simulink model "powertrain_model"  (R2025a)
settings: Solver=ode23tb  StartTime=0.0  StopTime=simlength  FixedStep=tc  MaxStep=tc
values from neighbouring files (symbols this model uses):
  angle_error = angle_error_deg/180*pi    (= 0)    [init_model.m]
  CTRPIFF_CLIP_RELEASE = 0.001    [init_model.m]
  dead_time = dead_time_INV    (= 4.2e-07)    [init_model.m]
  dead_time_INV = 0.42e-6    (= 4.2e-07)    [init_model.m]
  DThs_init = 0    [init_model.m]
  emf_fb_p = 0.2    [init_model.m]
  emf_fb_p_ccaller_1 = emf_fb_p    (= 0.2)    [init_model.m]
  emf_fb_p_ccaller_2 = emf_fb_p    (= 0.2)    [init_model.m]
  emf_p = emf_fb_p*4/10    (= 0.08)    [init_model.m]
  emf_p_ccaller_1 = emf_fb_p_ccaller_1*4/10    (= 0.08)    [init_model.m]
  emf_p_ccaller_2 = emf_fb_p_ccaller_2*4/10    (= 0.08)    [init_model.m]
  fPWM_INV = 25e3    (= 25000)    [init_model.m]
  g0_reference_flt = fcut_reference_flt * ts_inv * 2*pi    (= 0.00100530964915)    [init_model.m]
  g1_reference_flt = 1 - g0_reference_flt    (= 0.998994690351)    [init_model.m]
  id_ref_if_pu = iload_rms_ref*sqrt(2)/ibez    [init_model.m]
  kalman_omega = kw    [init_model.m]
  kalman_theta = kg    [init_model.m]
  kg = K(1)    [init_model.m]
  ki_id = 2    [analysis_cc.m]    (also in init_model.m = 9)
  ki_iq = 9    [init_model.m]
  ki_w = 1    [init_model.m]
  kp_id = 0.15    [analysis_cc.m]    (also in init_model.m = 0.25)
  kp_iq = 0.2    [init_model.m]
  kp_w = 1    [init_model.m]
  kw = K(2)    [init_model.m]
  luenberger_l1 = Klo(1)    [init_model.m]
  luenberger_l2 = Klo(2)    [init_model.m]
  luenberger_l3 = Klo(3)    [init_model.m]
  motorc_m_scale = 2/3*Vdc_bez/ubez    [init_model.m]
  number_of_cells = 100    [init_model.m]
  omega_flt_fcut = 10    [init_model.m]
  omega_flt_g0 = omega_flt_fcut * ts_inv * 2*pi    (= 0.00251327412287)    [init_model.m]
  omega_flt_g1 = 1 - omega_flt_g0    (= 0.997486725877)    [init_model.m]
  omega_ref_if_pu = 1200*2*pi/omega_bez    [init_model.m]
  phase_compensation_omega = 0    [init_model.m]
  pwm_out_lim = 1    [init_model.m]
  Q = 10    [init_model.m]
  q1Kalman = ts_inv^2    (= 1.6e-09)    [init_model.m]
  q2Kalman = ts_inv^1    (= 4e-05)    [init_model.m]
  q3Kalman = 0    [init_model.m]
  rKalman = 1    [init_model.m]
  Tambient = 1    [init_model.m]
  tc = ts_inv/200    (= 2e-07)    [init_model.m]
  time_init = 0.025    [init_model.m]
  torque_ref = 64/ibez*torque_mode    [init_model.m]
  ts_inv = 1/fPWM_INV    (= 4e-05)    [init_model.m]
  tsample = ts_inv    (= 4e-05)    [init_model.m]
  u_flt_g0 = u_flt_fcut * ts_inv * 2*pi    (= 0.904778684234)    [init_model.m]
  u_flt_g1 = 1 - u_flt_g0    (= 0.0952213157661)    [init_model.m]
  Vdc_bez = 400    [init_model.m]
undefined symbols (not defined in the file or in its folder): b, ibez, Jm, Jm_norm, Ld_norm, Lq_norm, Ls_norm, magnitude, omega_bez, psi_bez, psi_m, psi_m_norm, R_RLload, Rload_eq, Rs_norm, tau_bez, weigth
libraries: fl_lib x100, nesl_utility x84, ee_lib x11, cstblocks x4, lithium_ion_cell_lib x1, simulink x1, pmsm_uvw_with_harmonics_lib x1, pmsm_spatial_harmonics_uvw_lib x1, flexshaft_lib x1
(part 5 of 6)

== system powertrain_model/battery_system/battery_system/LithiumIonBattery/lithium ion cell analytical ocv/white_noise ==
  in : Inport
  Band-Limited White Noise : simulink/Sources/Band-Limited White Noise  Commented=on  Cov=tsample  Ts=tsample  seed=[23341]
  Sum2 : Sum  Inputs=|++
  out : Outport
  wires:
  Band-Limited White Noise/1 -> Sum2/2
  Sum2/1 -> out/1
  in/1 -> Sum2/1

== system powertrain_model/driver control/current_ctrl/vector_current_ctrl/dq_vector_pi/bounder1 ==
  md : Inport
  m_1 : Inport  Port=2
  m : Inport  Port=3
  Constant : Constant
  Constant1 : Constant  Value=0
  Divide : Product
  Switch : Switch  Threshold=pwm_out_lim  SaturateOnIntegerOverflow=off  InputSameDT=off
  Switch1 : Switch  Threshold=pwm_out_lim  SaturateOnIntegerOverflow=off  InputSameDT=off
  md_sat : Outport  VectorParamsAs1DForOutWhenUnconnected=off
  clip : Outport  Port=2  VectorParamsAs1DForOutWhenUnconnected=off
  wires:
  md/1 -> Switch1/3, Divide/2
  m_1/1 -> Divide/1
  Divide/1 -> Switch1/1
  Switch1/1 -> md_sat/1
  Switch/1 -> clip/1
  m/1 -> Switch/2, Switch1/2
  Constant/1 -> Switch/1
  Constant1/1 -> Switch/3

== system powertrain_model/driver control/current_ctrl/vector_current_ctrl/dq_vector_pi/bounder2 ==
  m : Inport
  m_1 : Inport  Port=2
  mq : Inport  Port=3
  Constant : Constant
  Constant1 : Constant  Value=0
  Divide : Product
  Switch : Switch  Threshold=pwm_out_lim  SaturateOnIntegerOverflow=off  InputSameDT=off
  Switch1 : Switch  Threshold=pwm_out_lim  SaturateOnIntegerOverflow=off  InputSameDT=off
  mq_sat : Outport  VectorParamsAs1DForOutWhenUnconnected=off
  clip : Outport  Port=2  VectorParamsAs1DForOutWhenUnconnected=off
  wires:
  Constant1/1 -> Switch/3
  Constant/1 -> Switch/1
  m/1 -> Switch1/2, Switch/2
  Switch/1 -> clip/1
  Switch1/1 -> mq_sat/1
  Divide/1 -> Switch1/1
  m_1/1 -> Divide/1
  mq/1 -> Divide/2, Switch1/3

== system powertrain_model/driver control/current_ctrl/vector_current_ctrl/dq_vector_pi/pi_d ==
  id_tilde : Inport
  clip : Inport  Port=2
  1/Ti : Gain  Gain=kp_id  SaturateOnIntegerOverflow=on  OutDataTypeStr=Inherit: Same as input  ParamDataTypeStr=Inherit: Same as input
  Constant : Constant  Value=0
  Constant1 : Constant  Value=Ls_norm
  Product : Product  Inputs=3
  Sum2 : Sum  Inputs=+-  SaturateOnIntegerOverflow=on
  Sum4 : Sum  SaturateOnIntegerOverflow=on
  Sum5 : Sum  Inputs=+++  SaturateOnIntegerOverflow=on
  Switch1 : Switch  Threshold=0.5  SaturateOnIntegerOverflow=off  InputSameDT=off
  Switch2 : Switch  Threshold=0.5  SaturateOnIntegerOverflow=off  InputSameDT=off
  Unit Delay1 : UnitDelay  SampleTime=ts_inv  HasFrameUpgradeWarning=on
  Unit Delay2 : UnitDelay  SampleTime=ts_inv  HasFrameUpgradeWarning=on
  kp1 : Gain  Gain=CTRPIFF_CLIP_RELEASE*ts_inv  SaturateOnIntegerOverflow=on  OutDataTypeStr=Inherit: Same as input  ParamDataTypeStr=Inherit: Same as input
  kp2 : Gain  Gain=ki_id*ts_inv  SaturateOnIntegerOverflow=on  OutDataTypeStr=Inherit: Same as input  ParamDataTypeStr=Inherit: Same as input
  kp3 : Gain  Gain=0  SaturateOnIntegerOverflow=on  OutDataTypeStr=Inherit: Same as input  ParamDataTypeStr=Inherit: Same as input
  ud_out : Outport  VectorParamsAs1DForOutWhenUnconnected=off
  wires:
  id_tilde/1 -> kp2/1, 1/Ti/1
  Switch1/1 -> Unit Delay2/1
  Sum4/1 -> Sum5/2, Switch1/3
  kp1/1 -> Sum2/2
  Sum2/1 -> Switch1/1
  Unit Delay2/1 -> Sum4/2, kp1/1, Sum2/1
  1/Ti/1 -> Sum5/1
  Switch2/1 -> Sum4/1
  kp2/1 -> Switch2/3
  clip/1 -> Unit Delay1/1
  [clip] -> Switch2/2
  [clip] -> Switch1/2
  Constant/1 -> Switch2/1
  Unit Delay1/1 -> [clip]
  Sum5/1 -> ud_out/1
  [iq_inverter_pu] -> Product/2
  [omega_pu_hat_flt] -> Product/1
  kp3/1 -> Sum5/3
  Constant1/1 -> Product/3
  Product/1 -> kp3/1

== system powertrain_model/driver control/current_ctrl/vector_current_ctrl/dq_vector_pi/pi_q ==
  iq_tilde : Inport
  clip : Inport  Port=2
  1/Ti : Gain  Gain=kp_iq  SaturateOnIntegerOverflow=on  OutDataTypeStr=Inherit: Same as input  ParamDataTypeStr=Inherit: Same as input
  Constant : Constant  Value=0
  Constant1 : Constant  Value=Ls_norm
  Product : Product  Inputs=3
  Sum2 : Sum  Inputs=+-  SaturateOnIntegerOverflow=on
  Sum4 : Sum  SaturateOnIntegerOverflow=on
  Sum5 : Sum  Inputs=+++  SaturateOnIntegerOverflow=on
  Switch1 : Switch  Threshold=0.5  SaturateOnIntegerOverflow=off  InputSameDT=off
  Switch2 : Switch  Threshold=0.5  SaturateOnIntegerOverflow=off  InputSameDT=off
  Unit Delay1 : UnitDelay  SampleTime=ts_inv  HasFrameUpgradeWarning=on
  Unit Delay2 : UnitDelay  SampleTime=ts_inv  HasFrameUpgradeWarning=on
  kp1 : Gain  Gain=CTRPIFF_CLIP_RELEASE*ts_inv  SaturateOnIntegerOverflow=on  OutDataTypeStr=Inherit: Same as input  ParamDataTypeStr=Inherit: Same as input
  kp2 : Gain  Gain=ki_iq*ts_inv  SaturateOnIntegerOverflow=on  OutDataTypeStr=Inherit: Same as input  ParamDataTypeStr=Inherit: Same as input
  kp3 : Gain  Gain=0  SaturateOnIntegerOverflow=on  OutDataTypeStr=Inherit: Same as input  ParamDataTypeStr=Inherit: Same as input
  Vqs_out : Outport  VectorParamsAs1DForOutWhenUnconnected=off
  wires:
  Constant/1 -> Switch2/1
  [clip] -> Switch1/2
  [clip] -> Switch2/2
  clip/1 -> Unit Delay1/1
  kp2/1 -> Switch2/3
  Switch2/1 -> Sum4/1
  1/Ti/1 -> Sum5/1
  Unit Delay2/1 -> Sum2/1, kp1/1, Sum4/2
  Sum2/1 -> Switch1/1
  kp1/1 -> Sum2/2
  Sum4/1 -> Sum5/2, Switch1/3
  Switch1/1 -> Unit Delay2/1
  iq_tilde/1 -> 1/Ti/1, kp2/1
  Unit Delay1/1 -> [clip]
  Sum5/1 -> Vqs_out/1
  [omega_pu_hat_flt] -> Product/1
  [id_inverter_pu] -> Product/2
  Constant1/1 -> Product/3
  Product/1 -> kp3/1
  kp3/1 -> Sum5/3

== system powertrain_model/driver control/current_ctrl/vector_current_ctrl/dq_vector_pi/switch ==
  clip 1 : Inport
  clip 2 : Inport  Port=2
  Constant4 : Constant
  Constant5 : Constant  Value=0
  Sum1 : Sum  SaturateOnIntegerOverflow=on
  Switch : Switch  Threshold=0.5  SaturateOnIntegerOverflow=off  InputSameDT=off
  clip : Outport  VectorParamsAs1DForOutWhenUnconnected=off
  wires:
  Constant5/1 -> Switch/3
  Switch/1 -> clip/1
  Constant4/1 -> Switch/1
  Sum1/1 -> Switch/2
  clip 1/1 -> Sum1/1
  clip 2/1 -> Sum1/2

== system powertrain_model/driver control/current_ctrl/vector_current_ctrl/dq_vector_pi/vector lenght ==
  md : Inport
  mq : Inport  Port=2
  Math Function : Math  Operator=magnitude^2  SignedPower=on
  Math Function1 : Math  Operator=magnitude^2  SignedPower=on
  Math Function2 : Math  Operator=reciprocal  SignedPower=on
  Sqrt : Sqrt
  Sum5 : Sum  SaturateOnIntegerOverflow=on
  m_1 : Outport  VectorParamsAs1DForOutWhenUnconnected=off
  m : Outport  Port=2  VectorParamsAs1DForOutWhenUnconnected=off
  wires:
  Sqrt/1 -> m/1, Math Function2/1
  mq/1 -> Math Function1/1
  Math Function1/1 -> Sum5/2
  Math Function/1 -> Sum5/1
  Sum5/1 -> Sqrt/1
  Math Function2/1 -> m_1/1
  md/1 -> Math Function/1

== system powertrain_model/driver control/current_ctrl/vector_current_ctrl/dq_vector_pi_ccaller/Reset Trigger ==
  Step : Step  Time=time_init  Before=1  After=0  SampleTime=0
  Out1 : Outport
  wires:
  Step/1 -> Out1/1  "Reset"

== system powertrain_model/inverter/MOS based inverter/inverter/inverter_mosfet_leg_thermal/mosfet_3 ==
  Diode : fl_lib/Electrical/Electrical Elements/Diode  Vf=Vgamma V  Ron=Ron Ohm  Goff=1e-8 1/Ohm  i_specify=off  i_priority=None  i=0 A  i_nominal_specify=off  i_nominal_value=1  i_nominal_unit=A  v_specify=off  v_priority=None  v=0 V  v_nominal_specify=off  v_nominal_value=1  v_nominal_unit=V
  Switch : fl_lib/Electrical/Electrical Elements/Switch  R_closed=Ron Ohm  G_open=1e-8 1/Ohm  Threshold=7.5  i_specify=off  i_priority=None  i=0 A  i_nominal_specify=off  i_nominal_value=1  i_nominal_unit=A  v_specify=off  v_priority=None  v=0 V  v_nominal_specify=off  v_nominal_value=1  v_nominal_unit=V
  G : PMIOPort  Side=Left
  C : PMIOPort  Port=2  Side=Left
  E : PMIOPort  Port=3  Side=Right
  connections:
  Diode/LConn1 -- E/RConn1 -- Switch/LConn1
  Switch/RConn1 -- G/RConn1
  Diode/RConn1 -- C/RConn1 -- Switch/RConn2

== system powertrain_model/inverter/MOS based inverter/inverter/inverter_mosfet_leg_thermal/mosfet_4 ==
  Diode : fl_lib/Electrical/Electrical Elements/Diode  Vf=Vgamma V  Ron=Ron Ohm  Goff=1e-8 1/Ohm  i_specify=off  i_priority=None  i=0 A  i_nominal_specify=off  i_nominal_value=1  i_nominal_unit=A  v_specify=off  v_priority=None  v=0 V  v_nominal_specify=off  v_nominal_value=1  v_nominal_unit=V
  Switch : fl_lib/Electrical/Electrical Elements/Switch  R_closed=Ron Ohm  G_open=1e-8 1/Ohm  Threshold=7.5  i_specify=off  i_priority=None  i=0 A  i_nominal_specify=off  i_nominal_value=1  i_nominal_unit=A  v_specify=off  v_priority=None  v=0 V  v_nominal_specify=off  v_nominal_value=1  v_nominal_unit=V
  G : PMIOPort  Side=Left
  C : PMIOPort  Port=2  Side=Left
  E : PMIOPort  Port=3  Side=Right
  connections:
  Switch/RConn2 -- C/RConn1 -- Diode/RConn1
  Switch/RConn1 -- G/RConn1
  Switch/LConn1 -- E/RConn1 -- Diode/LConn1

== system powertrain_model/inverter/MOS based inverter/inverter/inverter_mosfet_leg_thermal/mosfet_5 ==
  Diode : fl_lib/Electrical/Electrical Elements/Diode  Vf=Vgamma V  Ron=Ron Ohm  Goff=1e-8 1/Ohm  i_specify=off  i_priority=None  i=0 A  i_nominal_specify=off  i_nominal_value=1  i_nominal_unit=A  v_specify=off  v_priority=None  v=0 V  v_nominal_specify=off  v_nominal_value=1  v_nominal_unit=V
  Switch : fl_lib/Electrical/Electrical Elements/Switch  R_closed=Ron Ohm  G_open=1e-8 1/Ohm  Threshold=7.5  i_specify=off  i_priority=None  i=0 A  i_nominal_specify=off  i_nominal_value=1  i_nominal_unit=A  v_specify=off  v_priority=None  v=0 V  v_nominal_specify=off  v_nominal_value=1  v_nominal_unit=V
  G : PMIOPort  Side=Left
  C : PMIOPort  Port=2  Side=Left
  E : PMIOPort  Port=3  Side=Right
  connections:
  Diode/LConn1 -- E/RConn1 -- Switch/LConn1
  Switch/RConn1 -- G/RConn1
  Diode/RConn1 -- C/RConn1 -- Switch/RConn2

== system powertrain_model/inverter/MOS based inverter/inverter/inverter_mosfet_leg_thermal/mosfet_6 ==
  Diode : fl_lib/Electrical/Electrical Elements/Diode  Vf=Vgamma V  Ron=Ron Ohm  Goff=1e-8 1/Ohm  i_specify=off  i_priority=None  i=0 A  i_nominal_specify=off  i_nominal_value=1  i_nominal_unit=A  v_specify=off  v_priority=None  v=0 V  v_nominal_specify=off  v_nominal_value=1  v_nominal_unit=V
  Switch : fl_lib/Electrical/Electrical Elements/Switch  R_closed=Ron Ohm  G_open=1e-8 1/Ohm  Threshold=7.5  i_specify=off  i_priority=None  i=0 A  i_nominal_specify=off  i_nominal_value=1  i_nominal_unit=A  v_specify=off  v_priority=None  v=0 V  v_nominal_specify=off  v_nominal_value=1  v_nominal_unit=V
  G : PMIOPort  Side=Left
  C : PMIOPort  Port=2  Side=Left
  E : PMIOPort  Port=3  Side=Right
  connections:
  Switch/RConn2 -- C/RConn1 -- Diode/RConn1
  Switch/RConn1 -- G/RConn1
  Switch/LConn1 -- E/RConn1 -- Diode/LConn1

== system powertrain_model/inverter/MOS based inverter/inverter/inverter_mosfet_leg_thermal/mosfet_thermal_1 ==
  Heat Flow Rate Sensor : fl_lib/Thermal/Thermal Sensors/Heat Flow Rate Sensor
  MOSFET : ee_lib/Semiconductors & Converters/MOSFET (Ideal, Switching)  port_option=ee.enum.controlport.ps  Rds=Ron Ohm  Goff=1e-6 1/Ohm  Vth=7.5 V  diode_param=ee.enum.converters.protectiondiode.nodynamics  diode_Vf=Vgamma V  diode_Ron=0.001 Ohm  diode_Goff=1e-5 1/Ohm  diode_C=50e-9 F  diode_iRM=-235 A  diode_iF=300 A  diode_idot=-50 A/us  diode_trr_param=ee.enum.converters.diodeReverseParam.trr_factor  diode_trr_factor=3  diode_trr=15 us  diode_Qrr=1500 s*uA  ids_specify=off  ids_priority=None  ids=0 A  ids_nominal_specify=off  ids_nominal_value=1  ids_nominal_unit=A  vds_specify=off  vds_priority=None  vds=0 V  vds_nominal_specify=off  vds_nominal_value=1  vds_nominal_unit=V  vgs_specify=off  vgs_priority=None  vgs=0 V  vgs_nominal_specify=off  vgs_nominal_value=1  vgs_nominal_unit=V  thermal_loss_option=ee.enum.converters.thermalLossOption.constantvalues  Von_data=[0, 1.8, 3.2, 6, 10, 16; 0, 2, 5.5, 9.5, 15, 25] V  Tj=[298.15, 448.15] K  Iout_data=[0, 20, 40, 60, 80, 100] A  Eon_data=[0, 55.04, 124.57, 235.53, 362.12; 0, 71.25, 161.25, 304.88, 468.75] * 1e-6 J  Eoff_data=[0, 18, 30, 56.1, 76.5; 0, 22.5, 37.5, 70.13, 95.63] * 1e-6 J  Eon_data_3D=[zeros(2, 5, 3)] J  Eoff_data_3D=[zeros(2, 5, 3)] J  Tj_loss=[298.15, 448.15] K  Iout_data_loss=[0, 10, 20, 30, 40] A  tabulateWithVds=false  Vds_loss=[0, 150, 300] V  Eon_scalar=Eon J  Eoff_scalar=Eoff J  Voff=Voff_sw_losses V  Iout_scalar=Ion_sw_losses A  useCurrentFromPreviousCycle=true  useVoltageFromPreviousCycle=true  diodeModelType=ee.enum.converters.diodeModelType.pwl  diodeTableType=ee.enum.diode.tableType.IfMat  diode_ReverseIVType=ee.enum.diode.diodeReverseIV.constant  diode_IfMat=[.07, .12, .19, 1.75, 4.24, 7.32, 11.2; .16, .3, .72, 2.14, 4.02, 6.35, 9.12] A  diode_VfMat=[.9, 1.15, 1.25, 1.5, 1.75, 2.17, 2.6, 2.85; .58, .68, .75, 1.1, 1.38, 1.77, 2.27, 2.7] V  diode_TjVec=[25, 125] degC  diode_VfVec=[.5, .7, .9, 1.3, 1.7, 2.1, 2.5] V  diode_IfVec=[.1, .2, .5, 1, 2, 4, 7, 10] A  diode_IrMat=[1e-06, 2e-06, 5e-06, 1e-05, 2.5e-05, 5e-05, .0001; 2e-06, 5e-06, 1e-05, 4e-05, 8e-05, .0002, .0005] A  diode_VrMat=[10, 100, 200, 250, 300, 325, 350; 10, 70, 160, 220, 270, 300, 320] V  diode_VrVec=[10, 20, 40, 50, 70, 80, 100] V  diode_IrVec=[1e-06, 2e-06, 5e-06, 1e-05, 2e-05, 5e-05, .0001] A  diode_Vr=-600 V  diode_Ls=150 nH  diode_Erec=0.03 J  diode_rec_loss_model=ee.enum.diode.reverseRecoveryModel.fixed  diode_ErecVal=0 J  diode_scaleWithIandV=false  diode_ErecMat=zeros(2, 3) J  diode_TjrecVec=[298.15, 398.15] K  diode_IfrecVec=[.1, 1, 10] A  diode_IrecVal=10 A  diode_VrecVal=10 V  diode_tFilter=1 / 1000 / 100 s  separateThermalPortForDiode=false  thermal_network_parameterization=ee.enum.thermalNetworkTopology.external  Rth=[.03, .2] K/W  Rth_Cauer=[.03, .1, .2] K/W  Rth_Foster=[.03, .2] K/W  thermal_mass_parameterization=ee.enum.thermalNetwork.thermalmass  thermal_mass=[3, 25] J/K  thermal_mass_Cauer=[3, 10, 25] J/K  thermal_mass_Foster=[33, 50] J/K  thermal_time_constant=[.1, 5] s  thermal_time_constant_Cauer=[.1, 1, 5] s  thermal_time_constant_Foster=[1, 10] s  thermal_mass_initial_temperatures=[80, 80] degC  thermal_mass_initial_temperatures_Cauer=[25, 25, 25] degC  junction_thermal_mass=JunctionTermalMass J/K  Tvec_initial_Foster=[25, 25, 25, 25] degC  RthDiode=[.03, .2] K/W  RthCauerDiode=[.03, .1, .2] K/W  RthFosterDiode=[.03, .2] K/W  thermalMassDiode=[3, 25] J/K  thermalMassCauerDiode=[3, 10, 25] J/K  thermalMassFosterDiode=[33, 50] J/K  thermalTauDiode=[.1, 5] s  thermalTauCauerDiode=[.1, 1, 5] s  thermalTauFosterDiode=[1, 10] s  thermalMassInitTempDiode=[25, 25] degC  thermalMassInitTempCauerDiode=[25, 25, 25] degC  junctionthermalMassDiode=0.1 J/K  TVecInitialFosterDiode=[25, 25, 25, 25] degC  no_thermal_network=0  mosfet_junction_temperature_specify=on  mosfet_junction_temperature_priority=High  mosfet_junction_temperature=Tambient+DThs_init degC  mosfet_junction_temperature_nominal_specify=off  mosfet_junction_temperature_nominal_value=1  mosfet_junction_temperature_nominal_unit=degC  diode_junction_temperature_specify=off  diode_junction_temperature_priority=None  diode_junction_temperature=25 degC  diode_junction_temperature_nominal_specify=off  diode_junction_temperature_nominal_value=1  diode_junction_temperature_nominal_unit=degC  Qj_specify=off  Qj_priority=None  Qj=0 W  Qj_nominal_specify=off  Qj_nominal_value=1  Qj_nominal_unit=W  accumulatedSwitchingLosses_specify=off  accumulatedSwitchingLosses_priority=None  accumulatedSwitchingLosses=0 J
      settings: InternalSimscapePortConfiguration="{\"Bottom\":[],\"Left\":[{\"id\":\"G\",\"label\":\"\",\"type\":\"input\"},{\"id\":\"H\",\"label\":\"\",\"type\":\"foundation.thermal.thermal\"}],\"Right\":[{\"id\":\"D\",\"label\":\"\",\"type\":\"foundation.electrical.electrical\"},{\"id\":\"S\",\"label\":\"\",\"type\":\"foundation.electrical.electrical\"}],\"Top\":[]}"
  Mux : Mux  Inputs=2
  PS-Simulink Converter : nesl_utility/PS-Simulink Converter  PhysicalDomain=network_engine_domain  SubClassName=ps_output  LeftPortType=input  RightPortType=output  PseudoPeriodic=off  Frequencies=[]  VectorFormat=1-D array  Unit=W  AffineConversion=on
  PS-Simulink Converter1 : nesl_utility/PS-Simulink Converter  PhysicalDomain=network_engine_domain  SubClassName=ps_output  LeftPortType=input  RightPortType=output  PseudoPeriodic=off  Frequencies=[]  VectorFormat=1-D array  Unit=degC  AffineConversion=off
  PS-Simulink Converter2 : nesl_utility/PS-Simulink Converter  PhysicalDomain=network_engine_domain  SubClassName=ps_output  LeftPortType=input  RightPortType=output  PseudoPeriodic=off  Frequencies=[]  VectorFormat=1-D array  Unit=degC  AffineConversion=off
  Tambient : fl_lib/Thermal/Thermal Sources/Temperature Source  temperature=Tambient degC
  Temperature Sensor : fl_lib/Thermal/Thermal Sensors/Temperature Sensor  temperature_measure=foundation.enum.MeasurementReference.difference
  Temperature Sensor1 : fl_lib/Thermal/Thermal Sensors/Temperature Sensor  temperature_measure=foundation.enum.MeasurementReference.difference
  heatsink_C : fl_lib/Thermal/Thermal Elements/Thermal Mass  Commented=on  mass_type=foundation.enum.constant_variable.constant  mass=weigth/6 kg  sp_heat=cp_al J/(K*kg)  mass_min=1e-6 kg  num_ports=foundation.enum.numPorts2.one  m_specify=off  m_priority=High  m=1 kg  m_nominal_specify=off  m_nominal_value=1  m_nominal_unit=kg  T_specify=on  T_priority=High  T=DThs_init+Tambient degC  T_nominal_specify=off  T_nominal_value=1  T_nominal_unit=K  Q_specify=off  Q_priority=High  Q=0 W  Q_nominal_specify=off  Q_nominal_value=1  Q_nominal_unit=W
  heatsink_R : fl_lib/Thermal/Thermal Elements/Thermal Resistance  resistance=Rth_mosfet_HA K/W  T_specify=off  T_priority=High  T=0 deltadegC  T_nominal_specify=off  T_nominal_value=1  T_nominal_unit=K  Q_specify=off  Q_priority=None  Q=0 W  Q_nominal_specify=off  Q_nominal_value=1  Q_nominal_unit=W
  mosfet_sandwich : fl_lib/Thermal/Thermal Elements/Thermal Resistance  resistance=Rth_mosfet_JH K/W  T_specify=off  T_priority=High  T=0 degC  T_nominal_specify=off  T_nominal_value=1  T_nominal_unit=K  Q_specify=off  Q_priority=None  Q=0 W  Q_nominal_specify=off  Q_nominal_value=1  Q_nominal_unit=W
  power_losses_mosfet : Scope  NumInputPorts=2
      settings: SampleTime=tc  ActiveDisplayYMinimum=-4.643309447984473  ActiveDisplayYMaximum=41.789785031860546
  G : PMIOPort  Side=Left
  D : PMIOPort  Port=2  Side=Left
  S : PMIOPort  Port=3  Side=Right
  tag scope: mosfet_HA_temp=global, mosfet_JH_temp=global, mosfet_power_losses=global
  wires:
  PS-Simulink Converter/1 -> power_losses_mosfet/1, [mosfet_power_losses]  "Power Losses"
  PS-Simulink Converter2/1 -> [mosfet_HA_temp]  "mosfet_HA_temp"
  [mosfet_HA_temp] -> Mux/2
  PS-Simulink Converter1/1 -> [mosfet_JH_temp]  "mosfet_JH_temp"
  [mosfet_JH_temp] -> Mux/1
  Mux/1 -> power_losses_mosfet/2
  connections:
  D/RConn1 -- MOSFET/RConn1
  MOSFET/RConn2 -- S/RConn1
  G/RConn1 -- MOSFET/LConn1
  PS-Simulink Converter/LConn1 -- Heat Flow Rate Sensor/RConn1
  Temperature Sensor/LConn1 -- Heat Flow Rate Sensor/RConn2 -- mosfet_sandwich/LConn1
  mosfet_sandwich/RConn1 -- Temperature Sensor1/LConn1 -- Temperature Sensor/RConn1 -- heatsink_R/LConn1 -- heatsink_C/LConn1
  Temperature Sensor/RConn2 -- PS-Simulink Converter1/LConn1
  Tambient/LConn1 -- Temperature Sensor1/RConn1 -- heatsink_R/RConn1
  Temperature Sensor1/RConn2 -- PS-Simulink Converter2/LConn1
  MOSFET/LConn2 -- Heat Flow Rate Sensor/LConn1

== system powertrain_model/inverter/MOS based inverter/inverter/inverter_mosfet_leg_thermal/mosfet_thermal_2 ==
  MOSFET : ee_lib/Semiconductors & Converters/MOSFET (Ideal, Switching)  port_option=ee.enum.controlport.ps  Rds=Ron Ohm  Goff=1e-6 1/Ohm  Vth=7.5 V  diode_param=ee.enum.converters.protectiondiode.nodynamics  diode_Vf=Vgamma V  diode_Ron=0.001 Ohm  diode_Goff=1e-5 1/Ohm  diode_C=50e-9 F  diode_iRM=-235 A  diode_iF=300 A  diode_idot=-50 A/us  diode_trr_param=ee.enum.converters.diodeReverseParam.trr_factor  diode_trr_factor=3  diode_trr=15 us  diode_Qrr=1500 s*uA  ids_specify=off  ids_priority=None  ids=0 A  ids_nominal_specify=off  ids_nominal_value=1  ids_nominal_unit=A  vds_specify=off  vds_priority=None  vds=0 V  vds_nominal_specify=off  vds_nominal_value=1  vds_nominal_unit=V  vgs_specify=off  vgs_priority=None  vgs=0 V  vgs_nominal_specify=off  vgs_nominal_value=1  vgs_nominal_unit=V  thermal_loss_option=ee.enum.converters.thermalLossOption.constantvalues  Von_data=[0, 1.8, 3.2, 6, 10, 16; 0, 2, 5.5, 9.5, 15, 25] V  Tj=[298.15, 448.15] K  Iout_data=[0, 20, 40, 60, 80, 100] A  Eon_data=[0, 55.04, 124.57, 235.53, 362.12; 0, 71.25, 161.25, 304.88, 468.75] * 1e-6 J  Eoff_data=[0, 18, 30, 56.1, 76.5; 0, 22.5, 37.5, 70.13, 95.63] * 1e-6 J  Eon_data_3D=[zeros(2, 5, 3)] J  Eoff_data_3D=[zeros(2, 5, 3)] J  Tj_loss=[298.15, 448.15] K  Iout_data_loss=[0, 10, 20, 30, 40] A  tabulateWithVds=false  Vds_loss=[0, 150, 300] V  Eon_scalar=Eon J  Eoff_scalar=Eoff J  Voff=Voff_sw_losses V  Iout_scalar=Ion_sw_losses A  useCurrentFromPreviousCycle=true  useVoltageFromPreviousCycle=true  diodeModelType=ee.enum.converters.diodeModelType.pwl  diodeTableType=ee.enum.diode.tableType.IfMat  diode_ReverseIVType=ee.enum.diode.diodeReverseIV.constant  diode_IfMat=[.07, .12, .19, 1.75, 4.24, 7.32, 11.2; .16, .3, .72, 2.14, 4.02, 6.35, 9.12] A  diode_VfMat=[.9, 1.15, 1.25, 1.5, 1.75, 2.17, 2.6, 2.85; .58, .68, .75, 1.1, 1.38, 1.77, 2.27, 2.7] V  diode_TjVec=[25, 125] degC  diode_VfVec=[.5, .7, .9, 1.3, 1.7, 2.1, 2.5] V  diode_IfVec=[.1, .2, .5, 1, 2, 4, 7, 10] A  diode_IrMat=[1e-06, 2e-06, 5e-06, 1e-05, 2.5e-05, 5e-05, .0001; 2e-06, 5e-06, 1e-05, 4e-05, 8e-05, .0002, .0005] A  diode_VrMat=[10, 100, 200, 250, 300, 325, 350; 10, 70, 160, 220, 270, 300, 320] V  diode_VrVec=[10, 20, 40, 50, 70, 80, 100] V  diode_IrVec=[1e-06, 2e-06, 5e-06, 1e-05, 2e-05, 5e-05, .0001] A  diode_Vr=-600 V  diode_Ls=150 nH  diode_Erec=0.03 J  diode_rec_loss_model=ee.enum.diode.reverseRecoveryModel.fixed  diode_ErecVal=0 J  diode_scaleWithIandV=false  diode_ErecMat=zeros(2, 3) J  diode_TjrecVec=[298.15, 398.15] K  diode_IfrecVec=[.1, 1, 10] A  diode_IrecVal=10 A  diode_VrecVal=10 V  diode_tFilter=1 / 1000 / 100 s  separateThermalPortForDiode=false  thermal_network_parameterization=ee.enum.thermalNetworkTopology.external  Rth=[.03, .2] K/W  Rth_Cauer=[.03, .1, .2] K/W  Rth_Foster=[.03, .2] K/W  thermal_mass_parameterization=ee.enum.thermalNetwork.thermalmass  thermal_mass=[3, 25] J/K  thermal_mass_Cauer=[3, 10, 25] J/K  thermal_mass_Foster=[33, 50] J/K  thermal_time_constant=[.1, 5] s  thermal_time_constant_Cauer=[.1, 1, 5] s  thermal_time_constant_Foster=[1, 10] s  thermal_mass_initial_temperatures=[80, 80] degC  thermal_mass_initial_temperatures_Cauer=[25, 25, 25] degC  junction_thermal_mass=JunctionTermalMass J/K  Tvec_initial_Foster=[25, 25, 25, 25] degC  RthDiode=[.03, .2] K/W  RthCauerDiode=[.03, .1, .2] K/W  RthFosterDiode=[.03, .2] K/W  thermalMassDiode=[3, 25] J/K  thermalMassCauerDiode=[3, 10, 25] J/K  thermalMassFosterDiode=[33, 50] J/K  thermalTauDiode=[.1, 5] s  thermalTauCauerDiode=[.1, 1, 5] s  thermalTauFosterDiode=[1, 10] s  thermalMassInitTempDiode=[25, 25] degC  thermalMassInitTempCauerDiode=[25, 25, 25] degC  junctionthermalMassDiode=0.1 J/K  TVecInitialFosterDiode=[25, 25, 25, 25] degC  no_thermal_network=0  mosfet_junction_temperature_specify=on  mosfet_junction_temperature_priority=High  mosfet_junction_temperature=Tambient+DThs_init degC  mosfet_junction_temperature_nominal_specify=off  mosfet_junction_temperature_nominal_value=1  mosfet_junction_temperature_nominal_unit=degC  diode_junction_temperature_specify=off  diode_junction_temperature_priority=None  diode_junction_temperature=25 degC  diode_junction_temperature_nominal_specify=off  diode_junction_temperature_nominal_value=1  diode_junction_temperature_nominal_unit=degC  Qj_specify=off  Qj_priority=None  Qj=0 W  Qj_nominal_specify=off  Qj_nominal_value=1  Qj_nominal_unit=W  accumulatedSwitchingLosses_specify=off  accumulatedSwitchingLosses_priority=None  accumulatedSwitchingLosses=0 J
      settings: InternalSimscapePortConfiguration="{\"Bottom\":[],\"Left\":[{\"id\":\"G\",\"label\":\"\",\"type\":\"input\"},{\"id\":\"H\",\"label\":\"\",\"type\":\"foundation.thermal.thermal\"}],\"Right\":[{\"id\":\"D\",\"label\":\"\",\"type\":\"foundation.electrical.electrical\"},{\"id\":\"S\",\"label\":\"\",\"type\":\"foundation.electrical.electrical\"}],\"Top\":[]}"
  Tambient : fl_lib/Thermal/Thermal Sources/Temperature Source  temperature=Tambient degC
  heatsink_C : fl_lib/Thermal/Thermal Elements/Thermal Mass  Commented=on  mass_type=foundation.enum.constant_variable.constant  mass=weigth/6 kg  sp_heat=cp_al J/(K*kg)  mass_min=1e-6 kg  num_ports=foundation.enum.numPorts2.one  m_specify=off  m_priority=High  m=1 kg  m_nominal_specify=off  m_nominal_value=1  m_nominal_unit=kg  T_specify=on  T_priority=High  T=DThs_init+Tambient degC  T_nominal_specify=off  T_nominal_value=1  T_nominal_unit=K  Q_specify=off  Q_priority=High  Q=0 W  Q_nominal_specify=off  Q_nominal_value=1  Q_nominal_unit=W
  heatsink_R : fl_lib/Thermal/Thermal Elements/Thermal Resistance  resistance=Rth_mosfet_HA K/W  T_specify=off  T_priority=High  T=0 deltadegC  T_nominal_specify=off  T_nominal_value=1  T_nominal_unit=K  Q_specify=off  Q_priority=None  Q=0 W  Q_nominal_specify=off  Q_nominal_value=1  Q_nominal_unit=W
  mosfet_sandwich : fl_lib/Thermal/Thermal Elements/Thermal Resistance  resistance=Rth_mosfet_JH K/W  T_specify=off  T_priority=High  T=0 degC  T_nominal_specify=off  T_nominal_value=1  T_nominal_unit=K  Q_specify=off  Q_priority=None  Q=0 W  Q_nominal_specify=off  Q_nominal_value=1  Q_nominal_unit=W
  G : PMIOPort  Side=Left
  D : PMIOPort  Port=2  Side=Left
  S : PMIOPort  Port=3  Side=Right
  connections:
  mosfet_sandwich/LConn1 -- MOSFET/LConn2
  Tambient/LConn1 -- heatsink_R/RConn1
  heatsink_C/LConn1 -- heatsink_R/LConn1 -- mosfet_sandwich/RConn1
  G/RConn1 -- MOSFET/LConn1
  MOSFET/RConn2 -- S/RConn1
  D/RConn1 -- MOSFET/RConn1

== system powertrain_model/inverter/MOS based inverter/inverter/inverter_without_mosfet_leg_thermal/mosfet_1 ==
  Diode : fl_lib/Electrical/Electrical Elements/Diode  Vf=Vgamma V  Ron=Ron Ohm  Goff=1e-8 1/Ohm  i_specify=off  i_priority=None  i=0 A  i_nominal_specify=off  i_nominal_value=1  i_nominal_unit=A  v_specify=off  v_priority=None  v=0 V  v_nominal_specify=off  v_nominal_value=1  v_nominal_unit=V
  Switch : fl_lib/Electrical/Electrical Elements/Switch  R_closed=Ron Ohm  G_open=1e-8 1/Ohm  Threshold=7.5  i_specify=off  i_priority=None  i=0 A  i_nominal_specify=off  i_nominal_value=1  i_nominal_unit=A  v_specify=off  v_priority=None  v=0 V  v_nominal_specify=off  v_nominal_value=1  v_nominal_unit=V
  G : PMIOPort  Side=Left
  C : PMIOPort  Port=2  Side=Left
  E : PMIOPort  Port=3  Side=Right
  connections:
  Diode/LConn1 -- E/RConn1 -- Switch/LConn1
  Switch/RConn1 -- G/RConn1
  Diode/RConn1 -- C/RConn1 -- Switch/RConn2

== system powertrain_model/inverter/MOS based inverter/inverter/inverter_without_mosfet_leg_thermal/mosfet_2 ==
  Diode : fl_lib/Electrical/Electrical Elements/Diode  Vf=Vgamma V  Ron=Ron Ohm  Goff=1e-8 1/Ohm  i_specify=off  i_priority=None  i=0 A  i_nominal_specify=off  i_nominal_value=1  i_nominal_unit=A  v_specify=off  v_priority=None  v=0 V  v_nominal_specify=off  v_nominal_value=1  v_nominal_unit=V
  Switch : fl_lib/Electrical/Electrical Elements/Switch  R_closed=Ron Ohm  G_open=1e-8 1/Ohm  Threshold=7.5  i_specify=off  i_priority=None  i=0 A  i_nominal_specify=off  i_nominal_value=1  i_nominal_unit=A  v_specify=off  v_priority=None  v=0 V  v_nominal_specify=off  v_nominal_value=1  v_nominal_unit=V
  G : PMIOPort  Side=Left
  C : PMIOPort  Port=2  Side=Left
  E : PMIOPort  Port=3  Side=Right
  connections:
  Switch/RConn2 -- C/RConn1 -- Diode/RConn1
  Switch/RConn1 -- G/RConn1
  Switch/LConn1 -- E/RConn1 -- Diode/LConn1

== system powertrain_model/inverter/MOS based inverter/inverter/inverter_without_mosfet_leg_thermal/mosfet_3 ==
  Diode : fl_lib/Electrical/Electrical Elements/Diode  Vf=Vgamma V  Ron=Ron Ohm  Goff=1e-8 1/Ohm  i_specify=off  i_priority=None  i=0 A  i_nominal_specify=off  i_nominal_value=1  i_nominal_unit=A  v_specify=off  v_priority=None  v=0 V  v_nominal_specify=off  v_nominal_value=1  v_nominal_unit=V
  Switch : fl_lib/Electrical/Electrical Elements/Switch  R_closed=Ron Ohm  G_open=1e-8 1/Ohm  Threshold=7.5  i_specify=off  i_priority=None  i=0 A  i_nominal_specify=off  i_nominal_value=1  i_nominal_unit=A  v_specify=off  v_priority=None  v=0 V  v_nominal_specify=off  v_nominal_value=1  v_nominal_unit=V
  G : PMIOPort  Side=Left
  C : PMIOPort  Port=2  Side=Left
  E : PMIOPort  Port=3  Side=Right
  connections:
  Switch/RConn2 -- C/RConn1 -- Diode/RConn1
  Switch/RConn1 -- G/RConn1
  Switch/LConn1 -- E/RConn1 -- Diode/LConn1

== system powertrain_model/inverter/MOS based inverter/inverter/inverter_without_mosfet_leg_thermal/mosfet_4 ==
  Diode : fl_lib/Electrical/Electrical Elements/Diode  Vf=Vgamma V  Ron=Ron Ohm  Goff=1e-8 1/Ohm  i_specify=off  i_priority=None  i=0 A  i_nominal_specify=off  i_nominal_value=1  i_nominal_unit=A  v_specify=off  v_priority=None  v=0 V  v_nominal_specify=off  v_nominal_value=1  v_nominal_unit=V
  Switch : fl_lib/Electrical/Electrical Elements/Switch  R_closed=Ron Ohm  G_open=1e-8 1/Ohm  Threshold=7.5  i_specify=off  i_priority=None  i=0 A  i_nominal_specify=off  i_nominal_value=1  i_nominal_unit=A  v_specify=off  v_priority=None  v=0 V  v_nominal_specify=off  v_nominal_value=1  v_nominal_unit=V
  G : PMIOPort  Side=Left
  C : PMIOPort  Port=2  Side=Left
  E : PMIOPort  Port=3  Side=Right
  connections:
  Diode/LConn1 -- E/RConn1 -- Switch/LConn1
  Switch/RConn1 -- G/RConn1
  Diode/RConn1 -- C/RConn1 -- Switch/RConn2

== system powertrain_model/inverter/MOS based inverter/inverter/inverter_without_mosfet_leg_thermal/mosfet_5 ==
  Diode : fl_lib/Electrical/Electrical Elements/Diode  Vf=Vgamma V  Ron=Ron Ohm  Goff=1e-8 1/Ohm  i_specify=off  i_priority=None  i=0 A  i_nominal_specify=off  i_nominal_value=1  i_nominal_unit=A  v_specify=off  v_priority=None  v=0 V  v_nominal_specify=off  v_nominal_value=1  v_nominal_unit=V
  Switch : fl_lib/Electrical/Electrical Elements/Switch  R_closed=Ron Ohm  G_open=1e-8 1/Ohm  Threshold=7.5  i_specify=off  i_priority=None  i=0 A  i_nominal_specify=off  i_nominal_value=1  i_nominal_unit=A  v_specify=off  v_priority=None  v=0 V  v_nominal_specify=off  v_nominal_value=1  v_nominal_unit=V
  G : PMIOPort  Side=Left
  C : PMIOPort  Port=2  Side=Left
  E : PMIOPort  Port=3  Side=Right
  connections:
  Switch/RConn2 -- C/RConn1 -- Diode/RConn1
  Switch/RConn1 -- G/RConn1
  Switch/LConn1 -- E/RConn1 -- Diode/LConn1

== system powertrain_model/inverter/MOS based inverter/inverter/inverter_without_mosfet_leg_thermal/mosfet_6 ==
  Diode : fl_lib/Electrical/Electrical Elements/Diode  Vf=Vgamma V  Ron=Ron Ohm  Goff=1e-8 1/Ohm  i_specify=off  i_priority=None  i=0 A  i_nominal_specify=off  i_nominal_value=1  i_nominal_unit=A  v_specify=off  v_priority=None  v=0 V  v_nominal_specify=off  v_nominal_value=1  v_nominal_unit=V
  Switch : fl_lib/Electrical/Electrical Elements/Switch  R_closed=Ron Ohm  G_open=1e-8 1/Ohm  Threshold=7.5  i_specify=off  i_priority=None  i=0 A  i_nominal_specify=off  i_nominal_value=1  i_nominal_unit=A  v_specify=off  v_priority=None  v=0 V  v_nominal_specify=off  v_nominal_value=1  v_nominal_unit=V
  G : PMIOPort  Side=Left
  C : PMIOPort  Port=2  Side=Left
  E : PMIOPort  Port=3  Side=Right
  connections:
  Diode/LConn1 -- E/RConn1 -- Switch/LConn1
  Switch/RConn1 -- G/RConn1
  Diode/RConn1 -- C/RConn1 -- Switch/RConn2

== system powertrain_model/inverter/MOS based inverter/sv_pwm/modulator/PWM generator 1 ==
  m_index : Inport
  Constant : Constant  Value=dead_time*f*2
  Constant1 : Constant  Value=1.02
  Data Type Conversion1 : DataTypeConversion
  Data Type Conversion2 : DataTypeConversion
  Gain : Gain  Gain=1/(pi/2)
  Gain1 : Gain  Gain=1/2*0.98
  Hit Crossing : HitCross  ShowOutputPort=off
  Hit Crossing1 : HitCross  ShowOutputPort=off
  Relational Operator1 : RelationalOperator  Operator=<=  InputSameDT=off
  Relational Operator2 : RelationalOperator  Operator=<=  InputSameDT=off
  Saturation1 : Saturate  UpperLimit=m_up  LowerLimit=m_low
  Sine Wave : Sin  Frequency=f*2*pi  Phase=-pi/2+ph  SampleTime=0
  Sum : Sum  Inputs=|++  SaturateOnIntegerOverflow=on
  Sum1 : Sum  Inputs=-+|  SaturateOnIntegerOverflow=on
  Sum2 : Sum  Inputs=|++
  Trigonometric Function1 : Trigonometry  Operator=asin
  m1 : Outport
  m2 : Outport  Port=2
  wires:
  Relational Operator1/1 -> Data Type Conversion1/1
  m_index/1 -> Saturation1/1
  Data Type Conversion1/1 -> m1/1, Hit Crossing/1
  Relational Operator2/1 -> Data Type Conversion2/1
  Data Type Conversion2/1 -> m2/1, Hit Crossing1/1
  Constant/1 -> Sum/2, Sum1/1
  Saturation1/1 -> Sum/1, Sum1/2
  Sum/1 -> Relational Operator1/1
  Sum1/1 -> Relational Operator2/2
  Sine Wave/1 -> Trigonometric Function1/1
  Constant1/1 -> Sum2/2
  Trigonometric Function1/1 -> Gain/1
  Gain/1 -> Sum2/1
  Sum2/1 -> Gain1/1
  Gain1/1 -> Relational Operator2/1, Relational Operator1/2

== system powertrain_model/inverter/MOS based inverter/sv_pwm/modulator/PWM generator 2 ==
  m_index : Inport
  Constant : Constant  Value=dead_time*f*2
  Constant1 : Constant  Value=1.02
  Data Type Conversion1 : DataTypeConversion
  Data Type Conversion2 : DataTypeConversion
  Gain : Gain  Gain=1/(pi/2)
  Gain1 : Gain  Gain=1/2*0.98
  Hit Crossing : HitCross  ShowOutputPort=off
  Hit Crossing1 : HitCross  ShowOutputPort=off
  Relational Operator1 : RelationalOperator  Operator=<=  InputSameDT=off
  Relational Operator2 : RelationalOperator  Operator=<=  InputSameDT=off
  Saturation1 : Saturate  UpperLimit=m_up  LowerLimit=m_low
  Sine Wave : Sin  Frequency=f*2*pi  Phase=-pi/2+ph  SampleTime=0
  Sum : Sum  Inputs=|++  SaturateOnIntegerOverflow=on
  Sum1 : Sum  Inputs=-+|  SaturateOnIntegerOverflow=on
  Sum2 : Sum  Inputs=|++
  Trigonometric Function1 : Trigonometry  Operator=asin
  m1 : Outport
  m2 : Outport  Port=2
  wires:
  Gain1/1 -> Relational Operator1/2, Relational Operator2/1
  Sum2/1 -> Gain1/1
  Gain/1 -> Sum2/1
  Trigonometric Function1/1 -> Gain/1
  Constant1/1 -> Sum2/2
  Sine Wave/1 -> Trigonometric Function1/1
  Sum1/1 -> Relational Operator2/2
  Sum/1 -> Relational Operator1/1
  Saturation1/1 -> Sum1/2, Sum/1
  Constant/1 -> Sum1/1, Sum/2
  Data Type Conversion2/1 -> Hit Crossing1/1, m2/1
  Relational Operator2/1 -> Data Type Conversion2/1
  Data Type Conversion1/1 -> Hit Crossing/1, m1/1
  m_index/1 -> Saturation1/1
  Relational Operator1/1 -> Data Type Conversion1/1

== system powertrain_model/inverter/MOS based inverter/sv_pwm/modulator/PWM generator 3 ==
  m_index : Inport
  Constant : Constant  Value=dead_time*f*2
  Constant1 : Constant  Value=1.02
  Data Type Conversion1 : DataTypeConversion
  Data Type Conversion2 : DataTypeConversion
  Gain : Gain  Gain=1/(pi/2)
  Gain1 : Gain  Gain=1/2*0.98
  Hit Crossing : HitCross  ShowOutputPort=off
  Hit Crossing1 : HitCross  ShowOutputPort=off
  Relational Operator1 : RelationalOperator  Operator=<=  InputSameDT=off
  Relational Operator2 : RelationalOperator  Operator=<=  InputSameDT=off
  Saturation1 : Saturate  UpperLimit=m_up  LowerLimit=m_low
  Sine Wave : Sin  Frequency=f*2*pi  Phase=-pi/2+ph  SampleTime=0
  Sum : Sum  Inputs=|++  SaturateOnIntegerOverflow=on
  Sum1 : Sum  Inputs=-+|  SaturateOnIntegerOverflow=on
  Sum2 : Sum  Inputs=|++
  Trigonometric Function1 : Trigonometry  Operator=asin
  m1 : Outport
  m2 : Outport  Port=2
  wires:
  Relational Operator1/1 -> Data Type Conversion1/1
  m_index/1 -> Saturation1/1
  Data Type Conversion1/1 -> m1/1, Hit Crossing/1
  Relational Operator2/1 -> Data Type Conversion2/1
  Data Type Conversion2/1 -> m2/1, Hit Crossing1/1
  Constant/1 -> Sum/2, Sum1/1
  Saturation1/1 -> Sum/1, Sum1/2
  Sum/1 -> Relational Operator1/1
  Sum1/1 -> Relational Operator2/2
  Sine Wave/1 -> Trigonometric Function1/1
  Constant1/1 -> Sum2/2
  Trigonometric Function1/1 -> Gain/1
  Gain/1 -> Sum2/1
  Sum2/1 -> Gain1/1
  Gain1/1 -> Relational Operator2/1, Relational Operator1/2

== system powertrain_model/inverter/MOS based inverter/sv_pwm/modulator1/PWM generator 1 ==
  m_index : Inport
  Constant : Constant  Value=dead_time*f*2
  Constant1 : Constant  Value=1.02
  Data Type Conversion1 : DataTypeConversion
  Data Type Conversion2 : DataTypeConversion
  Gain : Gain  Gain=1/(pi/2)
  Gain1 : Gain  Gain=1/2*0.98
  Hit Crossing : HitCross  ShowOutputPort=off
  Hit Crossing1 : HitCross  ShowOutputPort=off
  Relational Operator1 : RelationalOperator  Operator=<=  InputSameDT=off
  Relational Operator2 : RelationalOperator  Operator=<=  InputSameDT=off
  Saturation1 : Saturate  UpperLimit=m_up  LowerLimit=m_low
  Sine Wave : Sin  Frequency=f*2*pi  Phase=-pi/2+ph  SampleTime=0
  Sum : Sum  Inputs=|++  SaturateOnIntegerOverflow=on
  Sum1 : Sum  Inputs=-+|  SaturateOnIntegerOverflow=on
  Sum2 : Sum  Inputs=|++
  Trigonometric Function1 : Trigonometry  Operator=asin
  m1 : Outport
  m2 : Outport  Port=2
  wires:
  Gain1/1 -> Relational Operator1/2, Relational Operator2/1
  Sum2/1 -> Gain1/1
  Gain/1 -> Sum2/1
  Trigonometric Function1/1 -> Gain/1
  Constant1/1 -> Sum2/2
  Sine Wave/1 -> Trigonometric Function1/1
  Sum1/1 -> Relational Operator2/2
  Sum/1 -> Relational Operator1/1
  Saturation1/1 -> Sum1/2, Sum/1
  Constant/1 -> Sum1/1, Sum/2
  Data Type Conversion2/1 -> Hit Crossing1/1, m1/1
  Relational Operator2/1 -> Data Type Conversion2/1
  Data Type Conversion1/1 -> Hit Crossing/1, m2/1
  m_index/1 -> Saturation1/1
  Relational Operator1/1 -> Data Type Conversion1/1

== system powertrain_model/inverter/MOS based inverter/sv_pwm/modulator1/PWM generator 2 ==
  m_index : Inport
  Constant : Constant  Value=dead_time*f*2
  Constant1 : Constant  Value=1.02
  Data Type Conversion1 : DataTypeConversion
  Data Type Conversion2 : DataTypeConversion
  Gain : Gain  Gain=1/(pi/2)
  Gain1 : Gain  Gain=1/2*0.98
  Hit Crossing : HitCross  ShowOutputPort=off
  Hit Crossing1 : HitCross  ShowOutputPort=off
  Relational Operator1 : RelationalOperator  Operator=<=  InputSameDT=off
  Relational Operator2 : RelationalOperator  Operator=<=  InputSameDT=off
  Saturation1 : Saturate  UpperLimit=m_up  LowerLimit=m_low
  Sine Wave : Sin  Frequency=f*2*pi  Phase=-pi/2+ph  SampleTime=0
  Sum : Sum  Inputs=|++  SaturateOnIntegerOverflow=on
  Sum1 : Sum  Inputs=-+|  SaturateOnIntegerOverflow=on
  Sum2 : Sum  Inputs=|++
  Trigonometric Function1 : Trigonometry  Operator=asin
  m1 : Outport
  m2 : Outport  Port=2
  wires:
  Relational Operator1/1 -> Data Type Conversion1/1
  m_index/1 -> Saturation1/1
  Data Type Conversion1/1 -> m2/1, Hit Crossing/1
  Relational Operator2/1 -> Data Type Conversion2/1
  Data Type Conversion2/1 -> m1/1, Hit Crossing1/1
  Constant/1 -> Sum/2, Sum1/1
  Saturation1/1 -> Sum/1, Sum1/2
  Sum/1 -> Relational Operator1/1
  Sum1/1 -> Relational Operator2/2
  Sine Wave/1 -> Trigonometric Function1/1
  Constant1/1 -> Sum2/2
  Trigonometric Function1/1 -> Gain/1
  Gain/1 -> Sum2/1
  Sum2/1 -> Gain1/1
  Gain1/1 -> Relational Operator2/1, Relational Operator1/2

== system powertrain_model/inverter/MOS based inverter/sv_pwm/modulator1/PWM generator 3 ==
  m_index : Inport
  Constant : Constant  Value=dead_time*f*2
  Constant1 : Constant  Value=1.02
  Data Type Conversion1 : DataTypeConversion
  Data Type Conversion2 : DataTypeConversion
  Gain : Gain  Gain=1/(pi/2)
  Gain1 : Gain  Gain=1/2*0.98
  Hit Crossing : HitCross  ShowOutputPort=off
  Hit Crossing1 : HitCross  ShowOutputPort=off
  Relational Operator1 : RelationalOperator  Operator=<=  InputSameDT=off
  Relational Operator2 : RelationalOperator  Operator=<=  InputSameDT=off
  Saturation1 : Saturate  UpperLimit=m_up  LowerLimit=m_low
  Sine Wave : Sin  Frequency=f*2*pi  Phase=-pi/2+ph  SampleTime=0
  Sum : Sum  Inputs=|++  SaturateOnIntegerOverflow=on
  Sum1 : Sum  Inputs=-+|  SaturateOnIntegerOverflow=on
  Sum2 : Sum  Inputs=|++
  Trigonometric Function1 : Trigonometry  Operator=asin
  m1 : Outport
  m2 : Outport  Port=2
  wires:
  Gain1/1 -> Relational Operator1/2, Relational Operator2/1
  Sum2/1 -> Gain1/1
  Gain/1 -> Sum2/1
  Trigonometric Function1/1 -> Gain/1
  Constant1/1 -> Sum2/2
  Sine Wave/1 -> Trigonometric Function1/1
  Sum1/1 -> Relational Operator2/2
  Sum/1 -> Relational Operator1/1
  Saturation1/1 -> Sum1/2, Sum/1
  Constant/1 -> Sum1/1, Sum/2
  Data Type Conversion2/1 -> Hit Crossing1/1, m1/1
  Relational Operator2/1 -> Data Type Conversion2/1
  Data Type Conversion1/1 -> Hit Crossing/1, m2/1
  m_index/1 -> Saturation1/1
  Relational Operator1/1 -> Data Type Conversion1/1

== matlab function powertrain_model/driver control/bemf_observer/bemf_observer_simulink/double_integrator_observer/bounder2 ==
  data: u input; y output
function y = bounder(u)
    
    u = -pi + mod(u+3*pi,2*pi);
    
    y = u;
end

== matlab function powertrain_model/battery_system/battery_system/LithiumIonBattery/SOC_estimator/Kalman_observer/lithium-ion battery model ==
  data: i input; SOC output; u output; ts input; Q input; l1 input; l2 input; l3 input; vout input; x output
function [SOC, u, x] = lithium_ion_battery(i,ts,Q,l1,l2,l3,vout)

    persistent z_po ir_po h_po vout_hat

    if isempty(z_po)
        ir_po = 0;
        h_po = 0;
        z_po = 0.35;        
    end
    
        R0 = 0.15;
        R = 0.15;
        C = 0.1;
        M = 125;
        E_1 = -1.031;
        E0 = 3.685;
        E1 = 0.2156;
        E2 = 0;
        E3 = 0;
        Elog = -0.05;
        alpha = 35;
        N = 100;
        
        z_pr = z_po - ts/Q*i ;
    
        ir_pr = exp(-ts/(R*C))*ir_po + (1-exp(-ts/(R*C)))*i;

        h_pr = exp(-abs(i)*ts/Q)*h_po - (1-exp(-abs(i)*ts/Q))*sign(i);
        
        OCV = E_1*exp(-z_pr*alpha) + E0 + E1*z_pr + E2*z_pr^2 + E3*z_pr^3 + Elog*log(1-z_pr+ts);
        
        vout_hat = OCV*N + M*h_pr - R*ir_pr - R0*i;
        
        z_po = z_pr + l1*(vout - vout_hat);
        ir_po = ir_pr + l2*(vout - vout_hat);
        h_po = h_pr + l3*(vout - vout_hat);
        u = vout_hat;
        
        x = [z_po; ir_po; h_po];

    SOC = z_po;
end

== matlab function powertrain_model/driver control/current_ctrl/current_transformation/alphabeta2dq ==
  data: alpha input; d output; beta input; phase input; q output
function [d,q] = alphabeta2dq(alpha,beta,phase)

    d  =  alpha*cos(phase) + beta*sin(phase);
    q = -alpha*sin(phase) + beta*cos(phase);

end

== matlab function powertrain_model/driver control/current_ctrl/current_transformation/uvw2alphabeta ==
  data: u input; alpha output; v input; w input; beta output
function [alpha,beta] = uvw2alphabeta(u,v,w)

alpha = 2/3*(u - 1/2*v - 1/2*w);
beta  = 2/3*(sqrt(3)/2*(v - w));

end

== matlab function powertrain_model/driver control/current_ctrl/dq2alphabeta ==
  data: d input; alpha output; q input; phase input; beta output
function [alpha,beta] = dq2alphabeta(d,q,phase)

    alpha  =  d*cos(phase) - q*sin(phase);
    beta = d*sin(phase) + q*cos(phase);

end

== matlab function powertrain_model/driver control/i//f references/bounder2 ==
  data: u input; y output
function y = bounder(u)
    
    y = -pi + mod(u+3*pi,2*pi);

end

== matlab function powertrain_model/inverter/Gyro based inverter/uvw2alphabeta ==
  data: alpha input; u output; beta input; v output; w output
function [u,v,w] = alphabeta2uvw(alpha,beta)

u  = alpha;
v  = -0.5*alpha+sqrt(3)/2*beta;
w  = -0.5*alpha-sqrt(3)/2*beta;

end

== matlab function powertrain_model/driver control/current_ctrl/dq2alphabeta1 ==
  data: d input; alpha output; q input; phase input; beta output
function [alpha,beta] = dq2alphabeta(d,q,phase)

    alpha  =  d*cos(phase) - q*sin(phase);
    beta = d*sin(phase) + q*cos(phase);

end

== matlab function powertrain_model/battery_system/battery_system/LithiumIonBattery/SOC_estimator/Kalman_observer/kalman_observer_gains ==
  data: i input; ts input; l1 output; z input; q1 input; q2 input; q3 input; r input; Q input; l2 output; l3 output
function [l1,l2,l3] = EKF(i,ts,z,q1,q2,q3,r,Q)

    persistent  p11 p12 p13 p21 p22 p23 p31 p32 p33

    if isempty(p11)
        p11 = q1;
        p12 = 0;
        p13 = 0;
        p21 = 0;
        p22 = q2;
        p23 = 0;
        p31 = 0;
        p32 = 0;
        p33 = q3;
    end
    R = 0.15;
    C = 10;
    M = 125;
    E_1 = -1.031;
    E1 = 0.2156;
    E2 = 0;
    E3 = 0;
    Elog = -0.05;
    alpha = 35;

    a11 = 1;
    a12 = 0;
    a13 = 0;
    a21 = 0;
    a22 = exp(-ts/(R*C));
    a23 = 0;
    a31 = 0;
    a32 = 0;
    a33 = abs(exp(-i*ts/Q));

    c1 = -alpha*E_1*abs(exp(-alpha*z)) + E1 + 2*E2*z + 3*E3*z^2 - Elog/(1-z+ts);
    c2 = -R;
    c3 = M;
    
    p11_pr = a11*(a11*p11 + a12*p21 + a13*p31) + a12*(a11*p12 + a12*p22 + a13*p32) + a13*(a11*p13 + a12*p23 + a13*p33) + q1;

    p12_pr = a21*(a11*p11 + a12*p21 + a13*p31) + a22*(a11*p12 + a12*p22 + a13*p32) + a23*(a11*p13 + a12*p23 + a13*p33);

    p13_pr = a31*(a11*p11 + a12*p21 + a13*p31) + a32*(a11*p12 + a12*p22 + a13*p32) + a33*(a11*p13 + a12*p23 + a13*p33);

    p21_pr = a11*(a21*p11 + a22*p21 + a23*p31) + a12*(a21*p12 + a22*p22 + a23*p32) + a13*(a21*p13 + a22*p23 + a23*p33);

    p22_pr = a21*(a21*p11 + a22*p21 + a23*p31) + a22*(a21*p12 + a22*p22 + a23*p32) + a23*(a21*p13 + a22*p23 + a23*p33) + q2;

    p23_pr = a31*(a21*p11 + a22*p21 + a23*p31) + a32*(a21*p12 + a22*p22 + a23*p32) + a33*(a21*p13 + a22*p23 + a23*p33);

    p31_pr = a11*(a31*p11 + a32*p21 + a33*p31) + a12*(a31*p12 + a32*p22 + a33*p32) + a13*(a31*p13 + a32*p23 + a33*p33);

    p32_pr = a21*(a31*p11 + a32*p21 + a33*p31) + a22*(a31*p12 + a32*p22 + a33*p32) + a23*(a31*p13 + a32*p23 + a33*p33);

    p33_pr = a31*(a31*p11 + a32*p21 + a33*p31) + a32*(a31*p12 + a32*p22 + a33*p32) + a33*(a31*p13 + a32*p23 + a33*p33) + q3;

    den = c1*(c1*p11 + c2*p21 + c3*p31) + c2*(c1*p12 + c2*p22 + c3*p32) + c3*(c1*p13 + c2*p23 + c3*p33) + r;
 
    l1 = (c1*p11 + c2*p12 + c3*p13)/den;
    l2 = (c1*p21 + c2*p22 + c3*p23)/den;
    l3 = (c1*p31 + c2*p32 + c3*p33)/den;
    
    p11 = (1 - c1*l1)*p11_pr - c2*l1*p21_pr - c3*l1*p31_pr;
    
    p12 = (1 - c1*l1)*p12_pr - c2*l1*p22_pr - c3*l1*p32_pr;
    
    p13 = (1 - c1*l1)*p13_pr - c2*l1*p23_pr - c3*l1*p33_pr;
    
    p21 = -c1*l2*p11_pr + (1 - c2*l2)*p21_pr - c3*l2*p31_pr;
    
    p22 = -c1*l2*p12_pr + (1 - c2*l2)*p22_pr - c3*l2*p32_pr;
    
    p23 = -c1*l2*p13_pr + (1 - c2*l2)*p23_pr - c3*l2*p33_pr;
    
    p31 = -c1*l3*p11_pr - c2*l3*p21_pr + (1 - c3*l3)*p31_pr;
    
    p32 = -c1*l3*p12_pr - c2*l3*p22_pr + (1 - c3*l3)*p32_pr;
    
    p33 = -c1*l3*p13_pr - c2*l3*p23_pr + (1 - c3*l3)*p33_pr;
end

== matlab function powertrain_model/driver control/bemf_observer/bemf_observer_simulink/double_integrator_observer/bounder1 ==
  data: u input; y output
function y = bounder(u)
    
    u = -pi + mod(u+3*pi,2*pi);
    
    y = u;
end
